simulink model "imu_pitch_cal_sim"  (Simulink 9.0)
settings: Solver=FixedStepDiscrete  StartTime=start_time  StopTime=stop_time  FixedStep=0.020  RelTol=1e-3  EnableMultiTasking=on
InitFcn:
  | imu_pitch_cal_sim_init
values from neighbouring files (symbols this model uses):
  imuX = WeighDebug_TOAeef_imu_accelX_t27    [extra_tip_sim_init.m]    (also in imu_pitch_cal_sim_init.m = WeighDebug_TOAeef_imu_accelX_t194)
  imuY = WeighDebug_TOAeef_imu_accelY_t27    [extra_tip_sim_init.m]    (also in imu_pitch_cal_sim_init.m = WeighDebug_TOAeef_imu_accelY_t194)
  imuZ = WeighDebug_TOAeef_imu_accelZ_t27    [extra_tip_sim_init.m]    (also in imu_pitch_cal_sim_init.m = WeighDebug_TOAeef_imu_accelZ_t194)
  liftAngle = WeighDebug_TOAlift_angle_t27    [extra_tip_sim_init.m]    (also in imu_pitch_cal_sim_init.m = WeighDebug_TOAlift_angle_t194)
  liftCylLength = WeighDebug_LiftCylNormLen_t27    [extra_tip_sim_init.m]    (also in imu_pitch_cal_sim_init.m = WeighDebug_LiftCylLenghtNorm_Val_t194)
  liftCylPress = WeighDebug_LiftCylPres_t27    [extra_tip_sim_init.m]    (also in imu_pitch_cal_sim_init.m = WeighDebug_LiftCylPres_t194)
  s1c1 = 515    [imu_pitch_cal_sim_init.m]
  s1c2 = 548    [imu_pitch_cal_sim_init.m]
  s1c3 = 579    [imu_pitch_cal_sim_init.m]
  s2c1 = s1c3 + 1    (= 580)    [imu_pitch_cal_sim_init.m]
  s2c2 = 616    [imu_pitch_cal_sim_init.m]
  s2c3 = 646    [imu_pitch_cal_sim_init.m]
  steerAng = WeighDebug_TOAsteering_angle_t27    [extra_tip_sim_init.m]    (also in imu_pitch_cal_sim_init.m = WeighDebug_TOAsteering_angle_t194)
  tiltExt = WeighDebug_TOAtilt_extension_t27    [extra_tip_sim_init.m]    (also in imu_pitch_cal_sim_init.m = WeighDebug_TOAtilt_extension_t194)
  tiltHePress = WeighDebug_TOAtilt_he_pressure_t27    [extra_tip_sim_init.m]    (also in imu_pitch_cal_sim_init.m = WeighDebug_TOAtilt_he_pressure_t194)
  tiltRePress = WeighDebug_TOAtilt_re_pressure_t27    [extra_tip_sim_init.m]    (also in imu_pitch_cal_sim_init.m = WeighDebug_TOAtilt_re_pressure_t194)
  time = t27    [extra_tip_sim_init.m]    (also in imu_pitch_cal_sim_init.m = t194)
  time2 = t27    [extra_tip_sim_init.m]    (also in imu_pitch_cal_sim_init.m = t194)
undefined symbols (not defined in the file or in its folder): g, timestep, toa_appNumber, toa_imu_lpf_cutoff_hz, toa_imuBasicOrient, toa_liftBoreDia, toa_tiltBoreDia, toa_tiltNumCyl, toa_tiltRodDia, toa_toolBcLength
libraries: simulink x10, simulink_extras x2, lib_CATutils_Filters_1Pole_LowPass x2, lib_CATutils_Override x1, lib_imuCal x1
settings Model: LogicAnalyzerSignalOrdering=5dd0029d-0573-49e1-b82a-316668c0f863,9c1653df-ca6c-4435-bc59-59c042f1a04b,b085631a-3729-4051-976c-78eb5fade8d3,7d46beec-13ab-48f4-a3cd-fd0effd7abe8,b6a03e28-23cb-43f9-a248-fda54d9653ab,a37efb6f-6706-4435-ba35-0122ce8219fd,a8a2ce2a-5a46-45c1-9d46-6a4d6193dbf9,5d366e23-9e16-40ab-92ec-e6241a047015,b6cb7851-fc42-42d8-ba93-f76abef1ebeb,7eca61fc-1cd1-4022-a45b-67ff63c6626d,6142d480-2c12-41e6-bc69-adb81a4771c4,b3c5c01d-7cb6-4bb7-bbe8-a848e78f78ed,24d79649-15d2-4718-8ed2-926b01c05a24,d8f024a4-d935-44db-a83c-243ca19a82d6,456d51b4-31c5-4d8b-9e4a-36f8ba5986a5,e5bf8900-4f4f-4702-ba55-200edadc7652,670c9483-bb58-4bfd-81ee-4bca25119f9a,78d642a3-b1b9-4e6b-84df-a8ec2d1c8fc5,fb89492d-1250-4bf5-972c-88d3c591c784,e773cc5f-bf5a-4589-b78e-aa1b72e66aaf,7a194ec3-8c67-49e0-a814-e64707b03eab,5e584c15-33ad-4c90-aebe-4c0d8ccecd57,a748872e-ecb8-4d69-a457-438b54df085b,bf746cf6-b149-4b19-87a9-88a499d409ce,04501ed4-9feb-42f8-8fc5-352602800299,46692b40-c2fd-4c0a-8a50-25bd1b341a8a,945a29ba-1fc8-4fc9-9c14-24f1e94ed818  MinMaxOverflowLogging=MinMaxAndOverflow  Creator=gulamhs  LastModifiedBy=CurriSD
settings DataIOCC: ExternalInput=[t,u]  SaveCompleteFinalSimState=on  SaveFormat=StructureWithTime  SaveOutput=off  SignalLogging=off  DSMLogging=off  SaveTime=off
settings OptimizationCC: DefaultParameterBehavior=Inlined  InlineInvariantSignals=on  EnhancedBackFolding=on  StrengthReduction=on  BitfieldContainerType=uchar_T  PassReuseOutputArgsAs=Individual arguments  ExpressionDepthLimit=2147483647  EfficientFloat2IntCast=on
settings DebuggingCC: SignalInfNanChecking=warning  SignalRangeChecking=error  ReadBeforeWriteMsg=EnableAllAsError  WriteAfterWriteMsg=EnableAllAsError  WriteAfterReadMsg=EnableAllAsError  AlgebraicLoopMsg=error  ArtificialAlgebraicLoopMsg=error  SaveWithDisabledLinksMsg=error  SaveWithParameterizedLinksMsg=error  UnderspecifiedInitializationDetection=Simplified  MergeDetectMultiDrivingBlocksExec=error  BlockPriorityViolationMsg=error  SolverPrmCheckMsg=error  InheritedTsInSrcMsg=none  TasksWithSamePriorityMsg=error  SigSpecEnsureSampleTimeMsg=error  CheckMatrixSingularityMsg=error  IntegerOverflowMsg=error  ParameterUnderflowMsg=error  ParameterPrecisionLossMsg=none  FixptConstUnderflowMsg=error  FixptConstOverflowMsg=error  UnderSpecifiedDataTypeMsg=error  FcnCallInpInsideContextMsg=warning  UnconnectedInputMsg=error  UnconnectedOutputMsg=error  UnconnectedLineMsg=error  SFcnCompatibilityMsg=error  FrameProcessingCompatibilityMsg=warning  UniqueDataStoreMsg=error  BusObjectLabelMismatch=error  RootOutportRequireBusObject=error  AssertControl=DisableAll  ModelReferenceIOMsg=error  ModelReferenceVersionMismatchMessage=warning  ModelReferenceIOMismatchMessage=error  UnknownTsInhSupMsg=error  ModelReferenceDataLoggingMessage=error  StateNameClashWarn=warning  SimStateInterfaceChecksumMismatchMsg=error  StrictBusMsg=ErrorOnBusTreatedAsVector  BusNameAdapt=ErrorWithoutRepair  NonBusSignalsTreatedAsBus=error  SFInvalidInputDataAccessInChartInitDiag=error  SFNoUnconditionalDefaultTransitionDiag=error  SFTransitionOutsideNaturalParentDiag=error  SFUnreachableExecutionPathDiag=error  SFUndirectedBroadcastEventsDiag=error  SFExecutionAtInitializationDiag=warning  IntegerSaturationMsg=error
settings HardwareCC: ProdBitPerLong=64  ProdBitPerPointer=64  ProdBitPerSizeT=64  ProdBitPerPtrDiffT=64  ProdLargestAtomicInteger=Integer  ProdLargestAtomicFloat=Float  ProdIntDivRoundTo=Zero  ProdEndianess=LittleEndian  ProdWordSize=64  ProdHWDeviceType=Intel->x86-64 (Linux 64)
settings ModelReferenceCC: ParallelModelReferenceMATLABWorkerInit=Load Top Model  PropagateSignalLabelsOutOfModel=on
settings SFSimCC: SimUserIncludeDirs=..\c_src  SFSimEcho=off  SimGenImportedTypeDefs=on  MATLABDynamicMemAlloc=off
settings SFSimCC: SimUserSources=|
  | ../c_src/tipoff_assist.c
  | ../c_src/tipoff_assist_950_14A_HL.c
  | ../c_src/tipoff_assist_950_14A_LOG.c
  | ../c_src/tipoff_assist_950_14A_STD.c
  | ../c_src/tipoff_assist_950_14A_Z_HL.c
  | ../c_src/tipoff_assist_950_14A_Z_LOG.c
  | ../c_src/tipoff_assist_950_14A_Z_STD.c
  | ../c_src/tipoff_assist_962_14A_HL.c
  | ../c_src/tipoff_assist_962_14A_LOG.c
  | ../c_src/tipoff_assist_962_14A_STD.c
  | ../c_src/tipoff_assist_962_14A_Z_HL.c
  | ../c_src/tipoff_assist_962_14A_Z_STD.c
  | ../c_src/tipoff_assist_966_14A_HL.c
  | ../c_src/tipoff_assist_966_14A_LOG.c
  | ../c_src/tipoff_assist_966_14A_STD.c
  | ../c_src/tipoff_assist_972_14A_HL.c
  | ../c_src/tipoff_assist_972_14A_STD.c
  | ../c_src/tipoff_assist_972_14A_SL.c
  | ../c_src/tipoff_assist_980_14A_BLK.c
  | ../c_src/tipoff_assist_980_14A_HL.c
  | ../c_src/tipoff_assist_980_14A_HVY.c
  | ../c_src/tipoff_assist_980_14A_LOG.c
  | ../c_src/tipoff_assist_980_14A_STD.c
  | ../c_src/tipoff_assist_982_14A_HL.c
  | ../c_src/tipoff_assist_982_14A_LOG.c
  | ../c_src/tipoff_assist_982_14A_STD.c
settings RTWCC: SystemTargetFile=cat_PkgArch.tlc  GenCodeOnly=on  GenerateMakefile=off  TemplateMakefile=cat_PkgArch_default_tmf  Description=R7a CAT Package Architecture Code Generation.  GenerateReport=on  RTWUseSimCustomCode=on  CustomInclude=..\c_src  CodeProfilingSaveOptions=AllData  GenerateTraceReport=on  GenerateTraceReportSl=on  GenerateTraceReportSf=on  GenerateTraceReportEml=on  GenerateWebview=on  GenerateCodeMetricsReport=on  GenerateCodeReplacementReport=on
settings RTWCC: CustomSource=|
  | ../c_src/tipoff_assist.c
  | ../c_src/tipoff_assist_950_14A_HL.c
  | ../c_src/tipoff_assist_950_14A_LOG.c
  | ../c_src/tipoff_assist_950_14A_STD.c
  | ../c_src/tipoff_assist_950_14A_Z_HL.c
  | ../c_src/tipoff_assist_950_14A_Z_LOG.c
  | ../c_src/tipoff_assist_950_14A_Z_STD.c
  | ../c_src/tipoff_assist_962_14A_HL.c
  | ../c_src/tipoff_assist_962_14A_LOG.c
  | ../c_src/tipoff_assist_962_14A_STD.c
  | ../c_src/tipoff_assist_962_14A_Z_HL.c
  | ../c_src/tipoff_assist_962_14A_Z_STD.c
  | ../c_src/tipoff_assist_966_14A_HL.c
  | ../c_src/tipoff_assist_966_14A_LOG.c
  | ../c_src/tipoff_assist_966_14A_STD.c
  | ../c_src/tipoff_assist_972_14A_HL.c
  | ../c_src/tipoff_assist_972_14A_STD.c
  | ../c_src/tipoff_assist_972_14A_SL.c
  | ../c_src/tipoff_assist_980_14A_BLK.c
  | ../c_src/tipoff_assist_980_14A_HL.c
  | ../c_src/tipoff_assist_980_14A_HVY.c
  | ../c_src/tipoff_assist_980_14A_LOG.c
  | ../c_src/tipoff_assist_980_14A_STD.c
  | ../c_src/tipoff_assist_982_14A_HL.c
  | ../c_src/tipoff_assist_982_14A_LOG.c
  | ../c_src/tipoff_assist_982_14A_STD.c
settings CodeAppCC: ForceParamTrailComments=on  IgnoreCustomStorageClasses=off  MaxIdLength=63  OperatorAnnotations=on  SimulinkDataObjDesc=on  SFDataObjDesc=on  MATLABFcnDesc=on  MangleLength=4  CustomSymbolStrType=$N$R$M  InsertBlockDesc=on  MATLABSourceComments=on  InternalIdentifier=Classic  ReqsInCode=on  UseSimReservedNames=on
settings STFCustomTargetCC: UtilityFuncGeneration=Shared location  MultiwordTypeDef=User defined  IncludeMdlTerminateFcn=off  CombineOutputUpdateFcns=on  SuppressErrorStatus=on  ERTCustomFileBanners=on  SupportAbsoluteTime=off  MultiInstanceERTCode=on  CodeInterfacePackaging=Reusable function  SupportComplex=off  SupportContinuousTime=off  SupportNonInlinedSFcns=off  RemoveResetFunc=on  SupportVariableSizeSignals=on  ParenthesesLevel=Maximum  MATLABClassNameForMDSCustomization=Simulink.SoftwareTarget.ERTCustomization  GRTInterface=off  GenerateSharedConstants=off  SystemTargetFile=cat_PkgArch.tlc
settings ERTTargetCC: UtilityFuncGeneration=Shared location  MultiwordTypeDef=User defined  MultiwordLength=2048  ParMdlRefBuildCompliant=off  CompOptLevelCompliant=off  ConcurrentExecutionCompliant=off  IncludeMdlTerminateFcn=off  SuppressErrorStatus=on  SupportAbsoluteTime=off  MultiInstanceERTCode=on  CodeInterfacePackaging=Reusable function  SupportComplex=off  SupportVariableSizeSignals=on  ParenthesesLevel=Maximum  ModelStepFunctionPrototypeControlCompliant=off  CPPClassGenCompliant=off  UseToolchainInfoCompliant=off  GenerateSharedConstants=off  MultiInstanceErrorCode=None  ERTSrcFileBannerTemplate=cat_code_template.cgt  ERTHdrFileBannerTemplate=cat_code_template.cgt  ERTDataSrcFileTemplate=cat_code_template.cgt  ERTDataHdrFileTemplate=cat_code_template.cgt  ERTCustomFileTemplate=cat_PkgArch_CFP.tlc  SuppressUnreachableDefaultCases=off  EnableUserReplacementTypes=on
settings MATStruct: int32=int32_t  int16=int16_t  int8=int8_t  uint32=uint32_t  uint16=uint16_t  uint8=uint8_t
settings CustomProperty: Value=Development
settings EnumStrPairs: String=Development
settings ConfigComp: CovScope=Subsystem  CovPath=/Chart1  CovMetricSettings=r  CovHtmlReporting=off  CovSaveCumulativeToWorkspaceVar=off  CovSaveSingleToWorkspaceVar=off  CovExternalEMLEnable=on

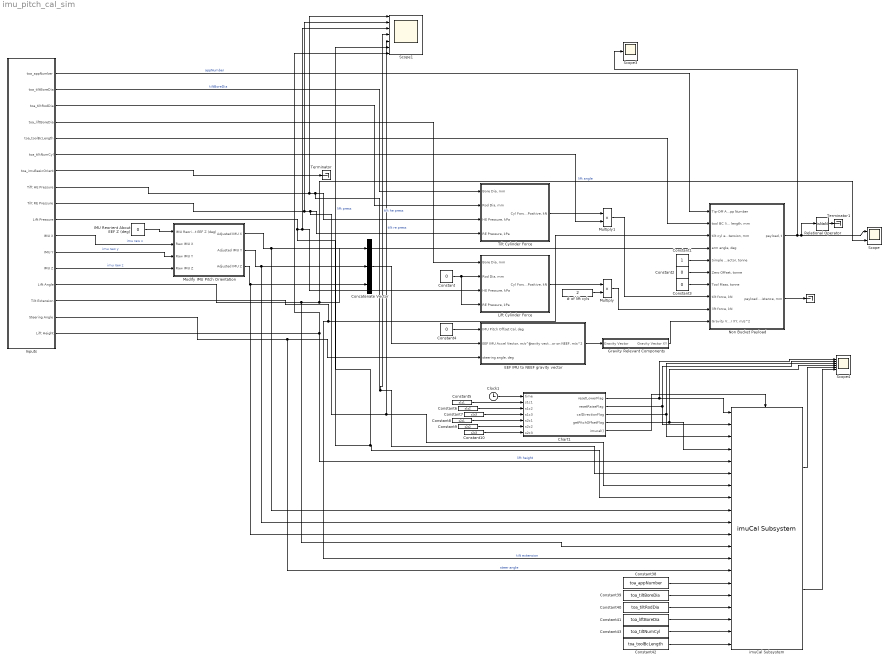
== system imu_pitch_cal_sim ==
  " " : Terminator
  # of lift cyls : Constant  Value=2  OutDataTypeStr=single
  Chart1 : Stateflow chart  TreatAsAtomicUnit=on
  Clock1 : Clock
      settings: Decimation=1000
  Concatenate Vector : Concatenate  NumInputs=3  Mode=Multidimensional array
  Constant : Constant  Value=0  OutDataTypeStr=Inherit: Inherit via back propagation
  Constant1 : Constant  OutDataTypeStr=single
  Constant10 : Constant  Value=s2c3
  Constant2 : Constant  Value=0  OutDataTypeStr=Inherit: Inherit via back propagation
  Constant3 : Constant  Value=0  OutDataTypeStr=Inherit: Inherit via back propagation
  Constant38 : Constant  Value=toa_appNumber  OutDataTypeStr=uint32
  Constant39 : Constant  Value=toa_tiltBoreDia  OutDataTypeStr=single
  Constant4 : Constant  Value=0  OutDataTypeStr=single
  Constant40 : Constant  Value=toa_tiltRodDia  OutDataTypeStr=single
  Constant41 : Constant  Value=toa_liftBoreDia  OutDataTypeStr=single
  Constant42 : Constant  Value=toa_toolBcLength  OutDataTypeStr=single
  Constant43 : Constant  Value=toa_tiltNumCyl  OutDataTypeStr=uint8
  Constant5 : Constant  Value=s1c1
  Constant6 : Constant  Value=s1c2
  Constant7 : Constant  Value=s1c3
  Constant8 : Constant  Value=s2c1
  Constant9 : Constant  Value=s2c2
  EEF IMU to NEEF gravity vector : Subsystem
  Gravity Relevant Components : Subsystem
  IMU Reorient About EEF Z (deg) : Constant  Value=0  OutDataTypeStr=single
  "Inputs " : Subsystem
  Lift Cylinder Force : Subsystem
  Modify IMU Pitch Orientation : Subsystem
  Multiply : Product  SaturateOnIntegerOverflow=on  RndMeth=Zero  InputSameDT=on  OutDataTypeStr=Inherit: Same as first input
  Multiply1 : Product  SaturateOnIntegerOverflow=on  RndMeth=Zero  InputSameDT=on  OutDataTypeStr=Inherit: Same as first input
  Non Bucket Payload : Subsystem
  Relational Operator : RelationalOperator  Operator=isNaN  OutDataTypeStr=boolean  RndMeth=Simplest
  Scope : Scope  NumInputPorts=2
  Scope1 : Scope  NumInputPorts=7
  Scope3 : Scope
  Scope4 : Scope  NumInputPorts=6
  Terminator : Terminator
  Terminator1 : Terminator
  Tilt Cylinder Force : Subsystem
  imuCal Subsystem : lib_imuCal/imuCal Subsystem
  wires:
  Multiply/1 -> Non Bucket Payload/9("lift force, kN")
  Non Bucket Payload/1("payload, t") -> Scope3/1, Scope/1, Relational Operator/1
  Multiply1/1 -> Non Bucket Payload/8("tilt force, kN")
  "Inputs "/6(toa_tiltNumCyl) -> Multiply1/2
  EEF IMU to NEEF gravity vector/1("gravity vector on NEEF, m/s^2") -> Gravity Relevant Components/1(Gravity Vector)
  Lift Cylinder Force/1("Cyl Force, Compression Positive, kN") -> Multiply/1
  Non Bucket Payload/2("payload distance, mm") -> " "/1
  # of lift cyls/1 -> Multiply/2
  Tilt Cylinder Force/1("Cyl Force, Compression Positive, kN") -> Multiply1/1
  Gravity Relevant Components/1(Gravity Vector XY) -> Non Bucket Payload/10("Gravity Vector XY, m/s^2")
  "Inputs "/1(toa_appNumber) -> Non Bucket Payload/1(Tip-Off Assist App Number)  "appNumber"
  "Inputs "/2(toa_tiltBoreDia) -> Tilt Cylinder Force/1("Bore Dia, mm")  "tiltBoreDia"
  "Inputs "/3(toa_tiltRodDia) -> Tilt Cylinder Force/2("Rod Dia, mm")
  "Inputs "/8(Tift HE Pressure) -> Scope1/1, Scope1/4, imuCal Subsystem/6, Tilt Cylinder Force/3("HE Pressure, kPa")  "tilt he press"
  "Inputs "/9(Tilt RE Pressure) -> Scope1/2, Scope1/5, imuCal Subsystem/7, Tilt Cylinder Force/4("RE Pressure, kPa")  "tilt re press"
  "Inputs "/4(toa_liftBoreDia) -> Lift Cylinder Force/1("Bore Dia, mm")
  "Inputs "/10(Lift Pressure) -> Scope1/6, imuCal Subsystem/8, Lift Cylinder Force/3("HE Pressure, kPa"), Scope1/3  "lift press"
  Constant/1 -> Lift Cylinder Force/4("RE Pressure, kPa"), Lift Cylinder Force/2("Rod Dia, mm")
  "Inputs "/11(IMU X) -> Modify IMU Pitch Orientation/2(Raw IMU X)  "imu raw x"
  Concatenate Vector/1 -> EEF IMU to NEEF gravity vector/2("EEF IMU Accel Vector, m/s^2")
  "Inputs "/16(Steering Angle) -> imuCal Subsystem/14, EEF IMU to NEEF gravity vector/3("steering angle, deg")  "steer angle"
  "Inputs "/15(Tilt Extension) -> imuCal Subsystem/13, Non Bucket Payload/3("tilt cyl extension, mm")  "tilt extension"
  "Inputs "/14(Lift Angle) -> imuCal Subsystem/12, Scope/2, Non Bucket Payload/4("arm angle, deg")  "lift angle"
  "Inputs "/7(toa_imuBasicOrient) -> Terminator/1
  "Inputs "/5(toa_toolBcLength) -> Non Bucket Payload/2("tool BC link length, mm")
  Constant1/1 -> Non Bucket Payload/5("Simple Cal Factor, tonne")
  Constant2/1 -> Non Bucket Payload/6("Zero Offset, tonne")
  Constant3/1 -> Non Bucket Payload/7("Tool Mass, tonne")
  Relational Operator/1 -> Terminator1/1
  Constant4/1 -> EEF IMU to NEEF gravity vector/1("IMU Pitch Offset Cal, deg")
  Chart1/1(resetLowerFlag) -> Scope4/1, imuCal Subsystem/1
  Chart1/3(calDirectionFlag) -> Scope4/3, imuCal Subsystem/3
  Chart1/4(getPitchOffsetFlag) -> Scope4/4, imuCal Subsystem/4
  Clock1/1 -> Chart1/1(time)
  "Inputs "/17(Lift Height) -> Scope1/7, imuCal Subsystem/5  "lift height"
  Chart1/2(resetRaiseFlag) -> Scope4/2, imuCal Subsystem/2
  Chart1/5(imucal()) -> imuCal Subsystem/Trigger
  imuCal Subsystem/1 -> Scope4/5
  Constant5/1 -> Chart1/2(s1c1)
  Constant6/1 -> Chart1/3(s1c2)
  Constant7/1 -> Chart1/4(s1c3)
  Constant8/1 -> Chart1/5(s2c1)
  Constant9/1 -> Chart1/6(s2c2)
  Constant10/1 -> Chart1/7(s2c3)
  Constant38/1 -> imuCal Subsystem/15
  Constant39/1 -> imuCal Subsystem/16
  Constant40/1 -> imuCal Subsystem/17
  Constant41/1 -> imuCal Subsystem/18
  Constant43/1 -> imuCal Subsystem/19
  Constant42/1 -> imuCal Subsystem/20
  IMU Reorient About EEF Z (deg)/1 -> Modify IMU Pitch Orientation/1(IMU Reorient EEF Z (deg))
  "Inputs "/12(IMU Y) -> Modify IMU Pitch Orientation/3(Raw IMU Y)  "imu raw y"
  "Inputs "/13(IMU Z) -> Modify IMU Pitch Orientation/4(Raw IMU Z)  "imu raw z"
  Modify IMU Pitch Orientation/1(Adjusted IMU X) -> imuCal Subsystem/9, Concatenate Vector/1
  Modify IMU Pitch Orientation/2(Adjusted IMU Y) -> imuCal Subsystem/10, Concatenate Vector/2
  Modify IMU Pitch Orientation/3(Adjusted IMU Z) -> imuCal Subsystem/11, Concatenate Vector/3
  imuCal Subsystem/2 -> Scope4/6

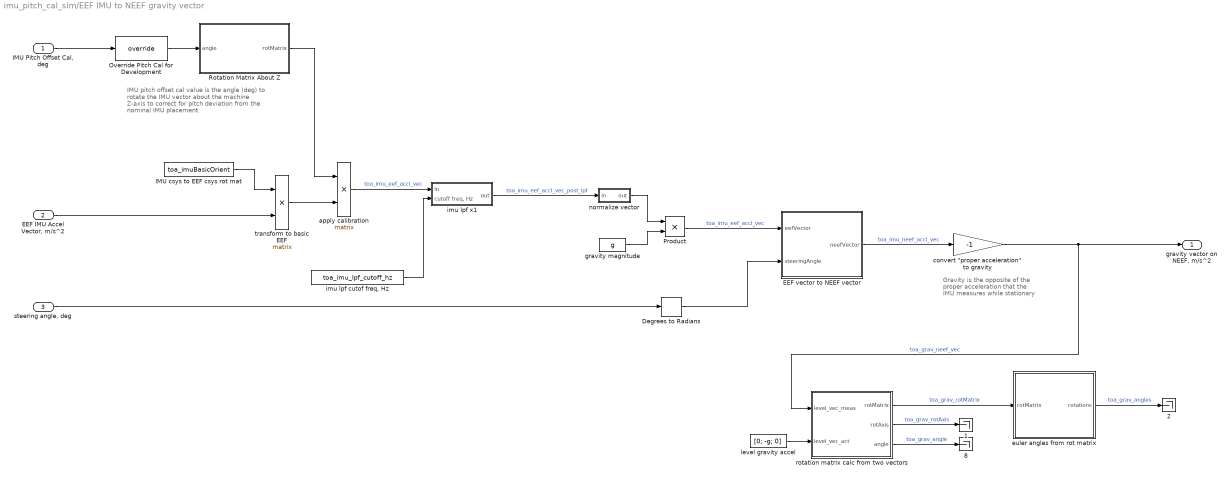
== system imu_pitch_cal_sim/EEF IMU to NEEF gravity vector ==
  note: Gravity is the opposite of the proper acceleration that the IMU measures while stationary
  note: IMU pitch offset cal value is the angle (deg) to rotate the IMU vector about the machine Z-axis to correct for pitch deviation from the nominal IMU placement.
  "IMU Pitch Offset Cal, deg" : Inport
  "EEF IMU Accel Vector, m/s^2" : Inport  Port=2
  "steering angle, deg" : Inport  Port=3
  " 1" : Terminator
  " 2" : Terminator
  " 8" : Terminator
  Degrees to Radians : simulink_extras/Transformations/Degrees to Radians
  EEF vector to NEEF vector : MATLAB Function  TreatAsAtomicUnit=on
  IMU csys to EEF csys rot mat : Constant  Value=toa_imuBasicOrient  VectorParams1D=off  OutDataTypeStr=single  SampleTime=-1
  Override Pitch Cal for Development : lib_CATutils_Override/override  ovType=OV if OV ~= Pass  extOV=off  ov_value=toa_imuCalPitchAngOv  extPass=off  pass_value=360  extRange=off  ov_max=100  ov_min=1  extCond=off  ov_cond=toa_imuCalPitchAngOv  extTF=off  ov_TrueComp=1  ov_FalseComp=2
  Product : Product  Inputs=**  OutDataTypeStr=Inherit: Same as first input
  Rotation Matrix About Z : MATLAB Function  TreatAsAtomicUnit=on
  apply calibration : Product  Multiplication=Matrix(*)  SaturateOnIntegerOverflow=on  RndMeth=Zero  OutDataTypeStr=Inherit: Same as first input
  "convert \"proper acceleration\" to gravity" : Gain  Gain=-1  SaturateOnIntegerOverflow=on  OutDataTypeStr=Inherit: Same as input  ParamDataTypeStr=Inherit: Same as input
  euler angles from rot matrix : MATLAB Function  TreatAsAtomicUnit=on
  gravity magnitude : Constant  Value=g  OutDataTypeStr=single  SampleTime=timestep
  "imu lpf cutof freq, Hz" : Constant  Value=toa_imu_lpf_cutoff_hz  OutDataTypeStr=single  SampleTime=timestep
  imu lpf x1 : Subsystem
  level gravity accel : Constant  Value=[0; -g; 0]  OutDataTypeStr=single  SampleTime=-1
  normalize vector : Subsystem
  rotation matrix calc from two vectors : MATLAB Function  TreatAsAtomicUnit=on
  transform to basic EEF : Product  Multiplication=Matrix(*)  SaturateOnIntegerOverflow=on  RndMeth=Zero  OutDataTypeStr=Inherit: Same as first input
  "gravity vector on NEEF, m/s^2" : Outport
  wires:
  "IMU Pitch Offset Cal, deg"/1 -> Override Pitch Cal for Development/1
  euler angles from rot matrix/1(rotations) -> " 2"/1  "toa_grav_angles"
  "imu lpf cutof freq, Hz"/1 -> imu lpf x1/2("cutoff freq, Hz")
  Degrees to Radians/1 -> EEF vector to NEEF vector/2(steeringAngle)
  Product/1 -> EEF vector to NEEF vector/1(eefVector)  "toa_imu_eef_accl_vec"
  "steering angle, deg"/1 -> Degrees to Radians/1
  EEF vector to NEEF vector/1(neefVector) -> "convert \"proper acceleration\" to gravity"/1  "toa_imu_neef_accl_vec"
  normalize vector/1(out) -> Product/1
  imu lpf x1/1(out) -> normalize vector/1(in)  "toa_imu_eef_accl_vec_post_lpf"
  gravity magnitude/1 -> Product/2
  Override Pitch Cal for Development/1 -> Rotation Matrix About Z/1(angle)
  Rotation Matrix About Z/1(rotMatrix) -> apply calibration/1
  apply calibration/1 -> imu lpf x1/1(in)  "toa_imu_eef_accl_vec"
  transform to basic EEF/1 -> apply calibration/2
  IMU csys to EEF csys rot mat/1 -> transform to basic EEF/1
  "convert \"proper acceleration\" to gravity"/1 -> rotation matrix calc from two vectors/1(level_vec_meas), "gravity vector on NEEF, m/s^2"/1  "toa_grav_neef_vec"
  "EEF IMU Accel Vector, m/s^2"/1 -> transform to basic EEF/2
  rotation matrix calc from two vectors/1(rotMatrix) -> euler angles from rot matrix/1(rotMatrix)  "toa_grav_rotMatrix"
  rotation matrix calc from two vectors/2(rotAxis) -> " 1"/1  "toa_grav_rotAxis"
  rotation matrix calc from two vectors/3(angle) -> " 8"/1  "toa_grav_angle"
  level gravity accel/1 -> rotation matrix calc from two vectors/2(level_vec_act)

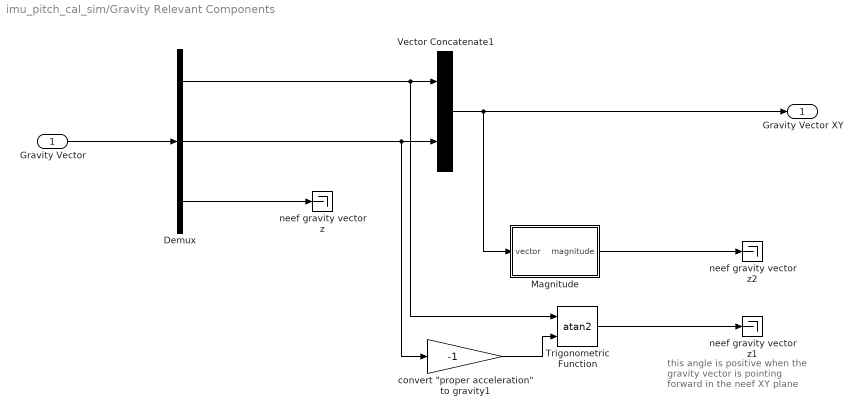
== system imu_pitch_cal_sim/Gravity Relevant Components ==
  note: this angle is positive when the gravity vector is pointing forward in the neef XY plane
  Gravity Vector : Inport
  " neef gravity vector z" : Terminator
  " neef gravity vector z1" : Terminator
  " neef gravity vector z2" : Terminator
  Demux : Demux  Outputs=3
  Magnitude : Subsystem
  Trigonometric Function : Trigonometry  Operator=atan2  OutputSignalType=real
  Vector Concatenate1 : Concatenate  Mode=Multidimensional array
  "convert \"proper acceleration\" to gravity1" : Gain  Gain=-1  SaturateOnIntegerOverflow=on  OutDataTypeStr=Inherit: Same as input  ParamDataTypeStr=Inherit: Same as input
  Gravity Vector XY : Outport
  wires:
  Gravity Vector/1 -> Demux/1
  Demux/2 -> "convert \"proper acceleration\" to gravity1"/1, Vector Concatenate1/2
  Demux/1 -> Trigonometric Function/1, Vector Concatenate1/1
  Magnitude/1(magnitude) -> " neef gravity vector z2"/1
  Trigonometric Function/1 -> " neef gravity vector z1"/1
  "convert \"proper acceleration\" to gravity1"/1 -> Trigonometric Function/2
  Demux/3 -> " neef gravity vector z"/1
  Vector Concatenate1/1 -> Magnitude/1(vector), Gravity Vector XY/1

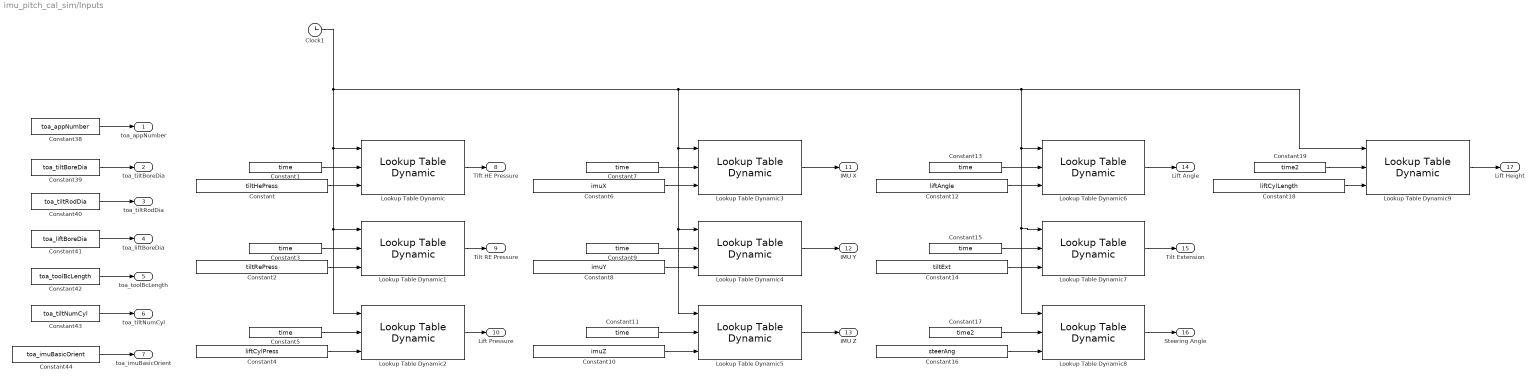
== system imu_pitch_cal_sim/Inputs  ==
  Clock1 : Clock
      settings: Decimation=1000
  Constant : Constant  Value=tiltHePress  SampleTime=timestep
  Constant{1,3,5,7,9,11,13,15} (8 alike) : Constant  Value=time  SampleTime=timestep
  Constant10 : Constant  Value=imuZ  SampleTime=timestep
  Constant12 : Constant  Value=liftAngle  SampleTime=timestep
  Constant14 : Constant  Value=tiltExt  SampleTime=timestep
  Constant16 : Constant  Value=steerAng  SampleTime=timestep
  Constant17 : Constant  Value=time2  SampleTime=timestep
  Constant18 : Constant  Value=liftCylLength  SampleTime=timestep
  Constant19 : Constant  Value=time2  SampleTime=timestep
  Constant2 : Constant  Value=tiltRePress  SampleTime=timestep
  Constant38 : Constant  Value=toa_appNumber  OutDataTypeStr=uint32
  Constant39 : Constant  Value=toa_tiltBoreDia  OutDataTypeStr=single
  Constant4 : Constant  Value=liftCylPress  SampleTime=timestep
  Constant40 : Constant  Value=toa_tiltRodDia  OutDataTypeStr=single
  Constant41 : Constant  Value=toa_liftBoreDia  OutDataTypeStr=single
  Constant42 : Constant  Value=toa_toolBcLength  OutDataTypeStr=single
  Constant43 : Constant  Value=toa_tiltNumCyl  OutDataTypeStr=single
  Constant44 : Constant  Value=toa_imuBasicOrient
  Constant6 : Constant  Value=imuX  SampleTime=timestep
  Constant8 : Constant  Value=imuY  SampleTime=timestep
  Lookup Table Dynamic{,1..9} (10 alike) : simulink/Lookup Tables/Lookup Table Dynamic  LookUpMeth=Interpolation-Use End Values  OutDataType=fixdt('single')  OutScaling=[]  OutputDataTypeScalingMode=Specify via dialog  OutDataTypeStr=single  DoSatur=off
      settings: SourceProductName=Simulink
  toa_appNumber : Outport  SampleTime=timestep
  toa_tiltBoreDia : Outport  Port=2  SampleTime=timestep
  toa_tiltRodDia : Outport  Port=3  SampleTime=timestep
  toa_liftBoreDia : Outport  Port=4  SampleTime=timestep
  toa_toolBcLength : Outport  Port=5  SampleTime=timestep
  toa_tiltNumCyl : Outport  Port=6  SampleTime=timestep
  toa_imuBasicOrient : Outport  Port=7  SampleTime=timestep
  Tift HE Pressure : Outport  Port=8  SampleTime=timestep
  Tilt RE Pressure : Outport  Port=9  SampleTime=timestep
  Lift Pressure : Outport  Port=10  SampleTime=timestep
  IMU X : Outport  Port=11  SampleTime=timestep
  IMU Y : Outport  Port=12  SampleTime=timestep
  IMU Z : Outport  Port=13  SampleTime=timestep
  Lift Angle : Outport  Port=14  SampleTime=timestep
  Tilt Extension : Outport  Port=15  SampleTime=timestep
  Steering Angle : Outport  Port=16  SampleTime=timestep
  Lift Height : Outport  Port=17  SampleTime=timestep
  wires:
  Constant17/1 -> Lookup Table Dynamic8/2
  Constant13/1 -> Lookup Table Dynamic6/2
  Lookup Table Dynamic6/1 -> Lift Angle/1
  Lookup Table Dynamic5/1 -> IMU Z/1
  Constant/1 -> Lookup Table Dynamic/3
  Lookup Table Dynamic2/1 -> Lift Pressure/1
  Constant3/1 -> Lookup Table Dynamic1/2
  Constant2/1 -> Lookup Table Dynamic1/3
  Constant8/1 -> Lookup Table Dynamic4/3
  Constant9/1 -> Lookup Table Dynamic4/2
  Constant12/1 -> Lookup Table Dynamic6/3
  Constant15/1 -> Lookup Table Dynamic7/2
  Lookup Table Dynamic7/1 -> Tilt Extension/1
  Lookup Table Dynamic8/1 -> Steering Angle/1
  Constant16/1 -> Lookup Table Dynamic8/3
  Constant11/1 -> Lookup Table Dynamic5/2
  Constant14/1 -> Lookup Table Dynamic7/3
  Constant6/1 -> Lookup Table Dynamic3/3
  Lookup Table Dynamic/1 -> Tift HE Pressure/1
  Constant4/1 -> Lookup Table Dynamic2/3
  Lookup Table Dynamic3/1 -> IMU X/1
  Lookup Table Dynamic4/1 -> IMU Y/1
  Constant1/1 -> Lookup Table Dynamic/2
  Constant7/1 -> Lookup Table Dynamic3/2
  Constant5/1 -> Lookup Table Dynamic2/2
  Constant10/1 -> Lookup Table Dynamic5/3
  Lookup Table Dynamic1/1 -> Tilt RE Pressure/1
  Constant39/1 -> toa_tiltBoreDia/1
  Constant38/1 -> toa_appNumber/1
  Constant40/1 -> toa_tiltRodDia/1
  Constant41/1 -> toa_liftBoreDia/1
  Constant42/1 -> toa_toolBcLength/1
  Constant43/1 -> toa_tiltNumCyl/1
  Constant44/1 -> toa_imuBasicOrient/1
  Clock1/1 -> Lookup Table Dynamic/1, Lookup Table Dynamic1/1, Lookup Table Dynamic2/1, Lookup Table Dynamic6/1, Lookup Table Dynamic7/1, Lookup Table Dynamic8/1, Lookup Table Dynamic9/1, Lookup Table Dynamic3/1, Lookup Table Dynamic5/1, Lookup Table Dynamic4/1
  Lookup Table Dynamic9/1 -> Lift Height/1
  Constant19/1 -> Lookup Table Dynamic9/2
  Constant18/1 -> Lookup Table Dynamic9/3

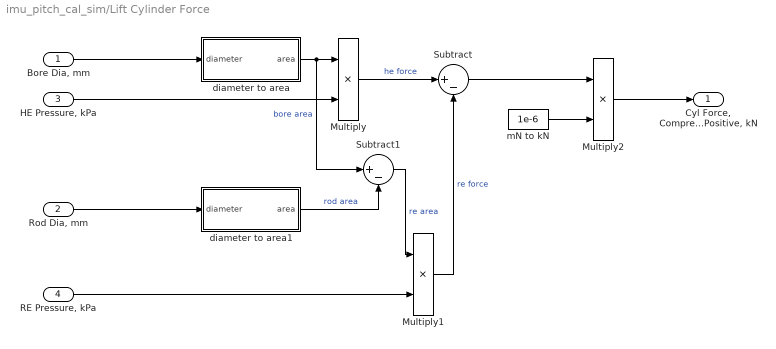
== system imu_pitch_cal_sim/Lift Cylinder Force ==
  "Bore Dia, mm" : Inport
  "Rod Dia, mm" : Inport  Port=2
  "HE Pressure, kPa" : Inport  Port=3
  "RE Pressure, kPa" : Inport  Port=4
  Multiply : Product  SaturateOnIntegerOverflow=on  RndMeth=Zero  InputSameDT=on  OutDataTypeStr=Inherit: Same as first input
  Multiply1 : Product  SaturateOnIntegerOverflow=on  RndMeth=Zero  InputSameDT=on  OutDataTypeStr=Inherit: Same as first input
  Multiply2 : Product  SaturateOnIntegerOverflow=on  RndMeth=Zero  InputSameDT=on  OutDataTypeStr=Inherit: Same as first input
  Subtract : Sum  Inputs=|+-  SaturateOnIntegerOverflow=on  InputSameDT=on  OutDataTypeStr=Inherit: Same as first input
  Subtract1 : Sum  Inputs=|+-  SaturateOnIntegerOverflow=on  InputSameDT=on  OutDataTypeStr=Inherit: Same as first input
  diameter to area : Subsystem
  diameter to area1 : Subsystem
  mN to kN : Constant  Value=1e-6  OutDataTypeStr=single
  "Cyl Force, Compression Positive, kN" : Outport
  wires:
  "HE Pressure, kPa"/1 -> Multiply/2
  Subtract/1 -> Multiply2/1
  "Bore Dia, mm"/1 -> diameter to area/1(diameter)
  Multiply1/1 -> Subtract/2  "re force"
  Multiply/1 -> Subtract/1  "he force"
  diameter to area/1(area) -> Subtract1/1, Multiply/1  "bore area"
  diameter to area1/1(area) -> Subtract1/2  "rod area"
  "RE Pressure, kPa"/1 -> Multiply1/2
  "Rod Dia, mm"/1 -> diameter to area1/1(diameter)
  Subtract1/1 -> Multiply1/1  "re area"
  mN to kN/1 -> Multiply2/2
  Multiply2/1 -> "Cyl Force, Compression Positive, kN"/1

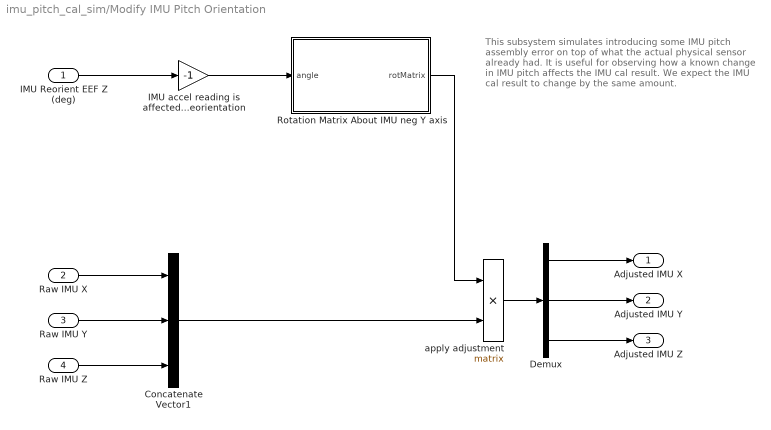
== system imu_pitch_cal_sim/Modify IMU Pitch Orientation ==
  note: This subsystem simulates introducing some IMU pitch assembly error on top of what the actual physical sensor already had. It is useful for observing how a known change in IMU pitch affects the IMU cal result. We expect the IMU cal result to change by the same amount.
  IMU Reorient EEF Z (deg) : Inport
  Raw IMU X : Inport  Port=2
  Raw IMU Y : Inport  Port=3
  Raw IMU Z : Inport  Port=4
  Concatenate Vector1 : Concatenate  NumInputs=3  Mode=Multidimensional array
  Demux : Demux  Outputs=3
  IMU accel reading is affected opposite of IMU body reorientation : Gain  Gain=-1
  Rotation Matrix About IMU neg Y axis : MATLAB Function  TreatAsAtomicUnit=on
  apply adjustment : Product  Multiplication=Matrix(*)  SaturateOnIntegerOverflow=on  RndMeth=Zero  OutDataTypeStr=Inherit: Same as first input
  Adjusted IMU X : Outport
  Adjusted IMU Y : Outport  Port=2
  Adjusted IMU Z : Outport  Port=3
  wires:
  Rotation Matrix About IMU neg Y axis/1(rotMatrix) -> apply adjustment/1
  apply adjustment/1 -> Demux/1
  Demux/1 -> Adjusted IMU X/1
  Demux/2 -> Adjusted IMU Y/1
  Demux/3 -> Adjusted IMU Z/1
  Raw IMU X/1 -> Concatenate Vector1/1
  Raw IMU Y/1 -> Concatenate Vector1/2
  IMU Reorient EEF Z (deg)/1 -> IMU accel reading is affected opposite of IMU body reorientation/1
  Raw IMU Z/1 -> Concatenate Vector1/3
  Concatenate Vector1/1 -> apply adjustment/2
  IMU accel reading is affected opposite of IMU body reorientation/1 -> Rotation Matrix About IMU neg Y axis/1(angle)

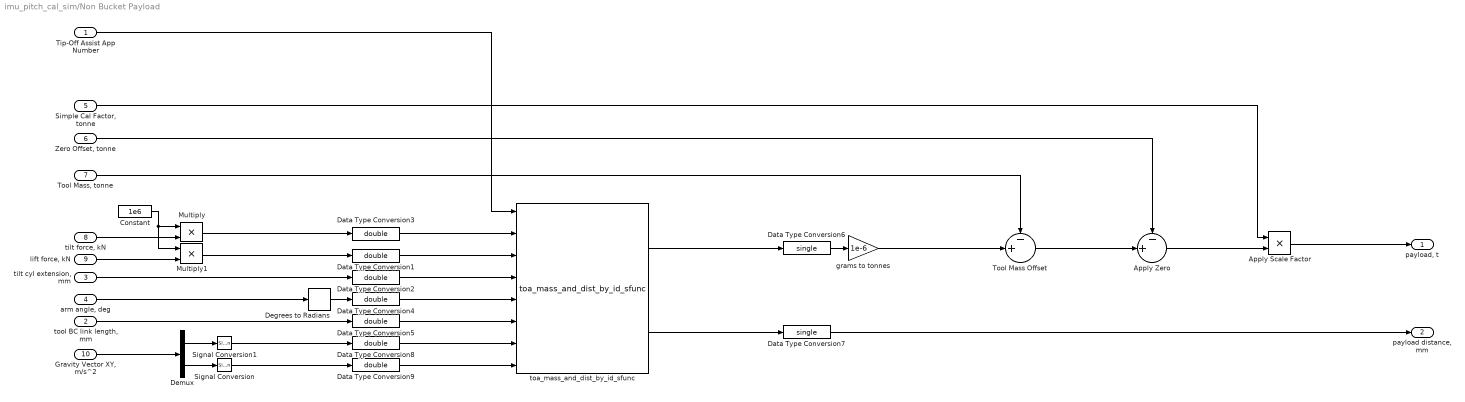
== system imu_pitch_cal_sim/Non Bucket Payload ==
  Tip-Off Assist App Number : Inport
  "tool BC link length, mm" : Inport  Port=2
  "tilt cyl extension, mm" : Inport  Port=3
  "arm angle, deg" : Inport  Port=4
  "Simple Cal Factor, tonne" : Inport  Port=5
  "Zero Offset, tonne" : Inport  Port=6
  "Tool Mass, tonne" : Inport  Port=7
  "tilt force, kN" : Inport  Port=8
  "lift force, kN" : Inport  Port=9
  "Gravity Vector XY, m/s^2" : Inport  Port=10
  Apply Scale Factor : Product
  Apply Zero : Sum  Inputs=-+|  SaturateOnIntegerOverflow=on  InputSameDT=on  OutDataTypeStr=Inherit: Same as first input
  Constant : Constant  Value=1e6  OutDataTypeStr=single
  Data Type Conversion{1..5,8..9} (7 alike) : DataTypeConversion  OutDataTypeStr=double  SaturateOnIntegerOverflow=on  RndMeth=Zero
      settings: AttributesFormatString=Output Data Type: %<OutDataTypeStr>\n
  Data Type Conversion6 : DataTypeConversion  OutDataTypeStr=single  SaturateOnIntegerOverflow=on  RndMeth=Zero
      settings: AttributesFormatString=Output Data Type: %<OutDataTypeStr>\n
  Data Type Conversion7 : DataTypeConversion  OutDataTypeStr=single  SaturateOnIntegerOverflow=on  RndMeth=Zero
      settings: AttributesFormatString=Output Data Type: %<OutDataTypeStr>\n
  Degrees to Radians : simulink_extras/Transformations/Degrees to Radians
  Demux : Demux  Outputs=2
  Multiply : Product  SaturateOnIntegerOverflow=on  RndMeth=Zero  InputSameDT=on  OutDataTypeStr=Inherit: Same as first input
  Multiply1 : Product  SaturateOnIntegerOverflow=on  RndMeth=Zero  InputSameDT=on  OutDataTypeStr=Inherit: Same as first input
  Signal Conversion : SignalConversion  OverrideOpt=on
  Signal Conversion1 : SignalConversion  OverrideOpt=on
  Tool Mass Offset : Sum  Inputs=-+|  SaturateOnIntegerOverflow=on  InputSameDT=on  OutDataTypeStr=Inherit: Same as first input
  grams to tonnes : Gain  Gain=1e-6  SaturateOnIntegerOverflow=on  OutDataTypeStr=Inherit: Same as input  ParamDataTypeStr=Inherit: Same as input
  toa_mass_and_dist_by_id_sfunc : S-Function  FunctionName=toa_mass_and_dist_by_id_sfunc  SFunctionDeploymentMode=off  EnableBusSupport=off  mask(Legacy Function){SFunctionSpec=void toa_mass_and_dist_by_id(uint32 u1, double u2, double u3, double u4, double u5, double u6, double u7, double u8, double y1[1], double y2[1]), ShowSpec=off}
      mask prompts: ShowSpec "Display function specification"
      mask help:
      | This block allows you to call the legacy functions specified by the following Legacy Code Tool definition:
      | def.SFunctionName = 'toa_mass_and_dist_by_id_sfunc';
      | def.OutputFcnSpec = 'void toa_mass_and_dist_by_id(uint32 u1, double u2, double u3, double u4, double u5, double u6, double u7, double u8, double y1[1], double y2[1])';
      | def.HeaderFiles = {'tipoff_assist.h'};
      | def.SourceFiles = {'tipoff_assist.c'};
      | def.IncPaths = {'./c_src'};
      mask Help: <p>This block was generated automatically by the Legacy Code Tool. For detailed help on this tool, call<a href="matlab:legacy_code('help')"> legacy_code('help')</a>.</p>
      mask Callback ShowSpec:
      | if strcmp(get_param(gcbh, 'ShowSpec'), 'on')
      |   set_param(gcbh, 'MaskDisplay', sprintf('fprintf(''%s'');', get_param(gcbh, 'SFunctionSpec')));
      | else
      |   set_param(gcbh, 'MaskDisplay', sprintf('fprintf(''%s'');', get_param(gcbh, 'FunctionName')));
      | end
      mask Display: fprintf('toa_mass_and_dist_by_id_sfunc');
  "payload, t" : Outport
  "payload distance, mm" : Outport  Port=2
  wires:
  Signal Conversion1/1 -> Data Type Conversion8/1
  Signal Conversion/1 -> Data Type Conversion9/1
  "tilt cyl extension, mm"/1 -> Data Type Conversion2/1
  Apply Scale Factor/1 -> "payload, t"/1
  Apply Zero/1 -> Apply Scale Factor/2
  "Simple Cal Factor, tonne"/1 -> Apply Scale Factor/1
  "Zero Offset, tonne"/1 -> Apply Zero/1
  Tool Mass Offset/1 -> Apply Zero/2
  Data Type Conversion3/1 -> toa_mass_and_dist_by_id_sfunc/2
  Data Type Conversion1/1 -> toa_mass_and_dist_by_id_sfunc/3
  Data Type Conversion2/1 -> toa_mass_and_dist_by_id_sfunc/4
  Data Type Conversion4/1 -> toa_mass_and_dist_by_id_sfunc/5
  Data Type Conversion5/1 -> toa_mass_and_dist_by_id_sfunc/6
  Data Type Conversion8/1 -> toa_mass_and_dist_by_id_sfunc/7
  Data Type Conversion9/1 -> toa_mass_and_dist_by_id_sfunc/8
  Tip-Off Assist App Number/1 -> toa_mass_and_dist_by_id_sfunc/1
  "tilt force, kN"/1 -> Multiply/2
  "lift force, kN"/1 -> Multiply1/2
  Constant/1 -> Multiply1/1, Multiply/1
  Data Type Conversion6/1 -> grams to tonnes/1
  Data Type Conversion7/1 -> "payload distance, mm"/1
  "Tool Mass, tonne"/1 -> Tool Mass Offset/1
  "Gravity Vector XY, m/s^2"/1 -> Demux/1
  grams to tonnes/1 -> Tool Mass Offset/2
  toa_mass_and_dist_by_id_sfunc/2 -> Data Type Conversion7/1
  toa_mass_and_dist_by_id_sfunc/1 -> Data Type Conversion6/1
  "tool BC link length, mm"/1 -> Data Type Conversion5/1
  Demux/2 -> Signal Conversion/1
  Demux/1 -> Signal Conversion1/1
  Multiply1/1 -> Data Type Conversion1/1
  Multiply/1 -> Data Type Conversion3/1
  "arm angle, deg"/1 -> Degrees to Radians/1
  Degrees to Radians/1 -> Data Type Conversion4/1

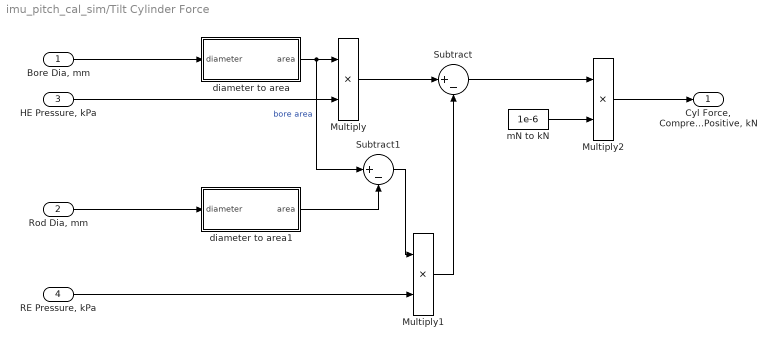
== system imu_pitch_cal_sim/Tilt Cylinder Force ==
  "Bore Dia, mm" : Inport
  "Rod Dia, mm" : Inport  Port=2
  "HE Pressure, kPa" : Inport  Port=3
  "RE Pressure, kPa" : Inport  Port=4
  Multiply : Product  SaturateOnIntegerOverflow=on  RndMeth=Zero  InputSameDT=on  OutDataTypeStr=Inherit: Same as first input
  Multiply1 : Product  SaturateOnIntegerOverflow=on  RndMeth=Zero  InputSameDT=on  OutDataTypeStr=Inherit: Same as first input
  Multiply2 : Product  SaturateOnIntegerOverflow=on  RndMeth=Zero  InputSameDT=on  OutDataTypeStr=Inherit: Same as first input
  Subtract : Sum  Inputs=|+-  SaturateOnIntegerOverflow=on  InputSameDT=on  OutDataTypeStr=Inherit: Same as first input
  Subtract1 : Sum  Inputs=|+-  SaturateOnIntegerOverflow=on  InputSameDT=on  OutDataTypeStr=Inherit: Same as first input
  diameter to area : Subsystem
  diameter to area1 : Subsystem
  mN to kN : Constant  Value=1e-6  OutDataTypeStr=single
  "Cyl Force, Compression Positive, kN" : Outport
  wires:
  "HE Pressure, kPa"/1 -> Multiply/2
  Subtract/1 -> Multiply2/1
  "Bore Dia, mm"/1 -> diameter to area/1(diameter)
  Multiply1/1 -> Subtract/2
  Multiply/1 -> Subtract/1
  diameter to area/1(area) -> Subtract1/1, Multiply/1  "bore area"
  diameter to area1/1(area) -> Subtract1/2
  "RE Pressure, kPa"/1 -> Multiply1/2
  "Rod Dia, mm"/1 -> diameter to area1/1(diameter)
  Subtract1/1 -> Multiply1/1
  mN to kN/1 -> Multiply2/2
  Multiply2/1 -> "Cyl Force, Compression Positive, kN"/1

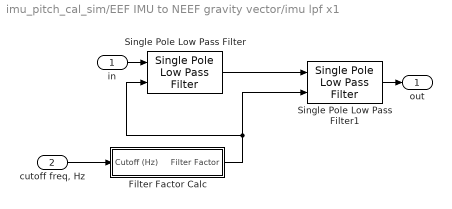
== system imu_pitch_cal_sim/EEF IMU to NEEF gravity vector/imu lpf x1 ==
  in : Inport
  "cutoff freq, Hz" : Inport  Port=2
  Filter Factor Calc : Subsystem
  Single Pole Low Pass Filter : lib_CATutils_Filters_1Pole_LowPass/Single Pole Low Pass Filter  extFactor=on  extReset=off  incIntWordSize=off  mainInternalRes=off  filtFactor=.0001
  Single Pole Low Pass Filter1 : lib_CATutils_Filters_1Pole_LowPass/Single Pole Low Pass Filter  extFactor=on  extReset=off  incIntWordSize=off  mainInternalRes=off  filtFactor=.0001
  out : Outport
  wires:
  Filter Factor Calc/1(Filter Factor) -> Single Pole Low Pass Filter/2, Single Pole Low Pass Filter1/2
  "cutoff freq, Hz"/1 -> Filter Factor Calc/1(Cutoff (Hz))
  Single Pole Low Pass Filter/1 -> Single Pole Low Pass Filter1/1
  Single Pole Low Pass Filter1/1 -> out/1
  in/1 -> Single Pole Low Pass Filter/1

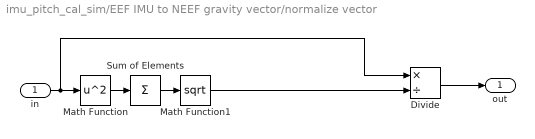
== system imu_pitch_cal_sim/EEF IMU to NEEF gravity vector/normalize vector ==
  in : Inport
  Divide : Product  Inputs=*/  OutDataTypeStr=Inherit: Same as first input
  Math Function : Math  Operator=square  SaturateOnIntegerOverflow=on
  Math Function1 : Math  Operator=sqrt  SaturateOnIntegerOverflow=on
  Sum of Elements : Sum  Inputs=+
  out : Outport
  wires:
  Sum of Elements/1 -> Math Function1/1
  Math Function/1 -> Sum of Elements/1
  Math Function1/1 -> Divide/2
  in/1 -> Divide/1, Math Function/1
  Divide/1 -> out/1

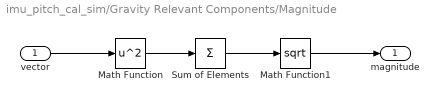
== system imu_pitch_cal_sim/Gravity Relevant Components/Magnitude ==
  vector : Inport
  Math Function : Math  Operator=square  SaturateOnIntegerOverflow=on
  Math Function1 : Math  Operator=sqrt  SaturateOnIntegerOverflow=on
  Sum of Elements : Sum  Inputs=+
  magnitude : Outport
  wires:
  Math Function1/1 -> magnitude/1
  Math Function/1 -> Sum of Elements/1
  Sum of Elements/1 -> Math Function1/1
  vector/1 -> Math Function/1

== system imu_pitch_cal_sim/Lift Cylinder Force/diameter to area ==
  diameter : Inport
  Constant2 : Constant  Value=pi/4  OutDataTypeStr=single
  Math Function : Math  Operator=square  OutputSignalType=real  SaturateOnIntegerOverflow=on
  Multiply2 : Product  SaturateOnIntegerOverflow=on  RndMeth=Zero  InputSameDT=on  OutDataTypeStr=Inherit: Same as first input
  area : Outport
  wires:
  Constant2/1 -> Multiply2/1
  Math Function/1 -> Multiply2/2
  Multiply2/1 -> area/1
  diameter/1 -> Math Function/1

== system imu_pitch_cal_sim/Lift Cylinder Force/diameter to area1 ==
  diameter : Inport
  Constant2 : Constant  Value=pi/4  OutDataTypeStr=single
  Math Function : Math  Operator=square  OutputSignalType=real  SaturateOnIntegerOverflow=on
  Multiply2 : Product  SaturateOnIntegerOverflow=on  RndMeth=Zero  InputSameDT=on  OutDataTypeStr=Inherit: Same as first input
  area : Outport
  wires:
  Constant2/1 -> Multiply2/1
  Math Function/1 -> Multiply2/2
  Multiply2/1 -> area/1
  diameter/1 -> Math Function/1

== system imu_pitch_cal_sim/Tilt Cylinder Force/diameter to area ==
  diameter : Inport
  Constant2 : Constant  Value=pi/4  OutDataTypeStr=single
  Math Function : Math  Operator=square  OutputSignalType=real  SaturateOnIntegerOverflow=on
  Multiply2 : Product  SaturateOnIntegerOverflow=on  RndMeth=Zero  InputSameDT=on  OutDataTypeStr=Inherit: Same as first input
  area : Outport
  wires:
  Constant2/1 -> Multiply2/1
  Math Function/1 -> Multiply2/2
  Multiply2/1 -> area/1
  diameter/1 -> Math Function/1

== system imu_pitch_cal_sim/Tilt Cylinder Force/diameter to area1 ==
  diameter : Inport
  Constant2 : Constant  Value=pi/4  OutDataTypeStr=single
  Math Function : Math  Operator=square  OutputSignalType=real  SaturateOnIntegerOverflow=on
  Multiply2 : Product  SaturateOnIntegerOverflow=on  RndMeth=Zero  InputSameDT=on  OutDataTypeStr=Inherit: Same as first input
  area : Outport
  wires:
  Constant2/1 -> Multiply2/1
  Math Function/1 -> Multiply2/2
  Multiply2/1 -> area/1
  diameter/1 -> Math Function/1

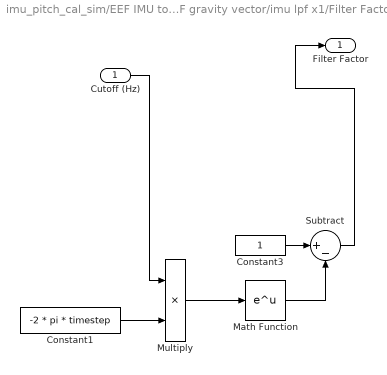
== system imu_pitch_cal_sim/EEF IMU to NEEF gravity vector/imu lpf x1/Filter Factor Calc ==
  Cutoff (Hz) : Inport
  Constant1 : Constant  Value=-2 * pi * timestep  OutDataTypeStr=single
  Constant3 : Constant  OutDataTypeStr=single
  Math Function : Math  OutputSignalType=real  SaturateOnIntegerOverflow=on
  Multiply : Product  SaturateOnIntegerOverflow=on  RndMeth=Zero  InputSameDT=on  OutDataTypeStr=Inherit: Same as first input
  Subtract : Sum  Inputs=|+-  SaturateOnIntegerOverflow=on  InputSameDT=on  OutDataTypeStr=Inherit: Same as first input
  Filter Factor : Outport
  wires:
  Constant1/1 -> Multiply/2
  Math Function/1 -> Subtract/2
  Multiply/1 -> Math Function/1
  Constant3/1 -> Subtract/1
  Subtract/1 -> Filter Factor/1
  Cutoff (Hz)/1 -> Multiply/1

== stateflow chart Chart1 ==
  state waitStart
  state raise
    en:
    calDirectionFlag = 0;
    resetRaiseFlag = 1;
    resetLowerFlag = 1;
    send(imucal)
    resetRaiseFlag = 0;
    resetLowerFlag = 0;
    du:
    send(imucal)
  state lower
    en:
    calDirectionFlag = 1;
    resetLowerFlag = 1;
    send(imucal)
    resetLowerFlag = 0;
    du:
    send(imucal)
  state endSet
    en:
    getPitchOffsetFlag = 1;
    send(imucal)
    ex:
    getPitchOffsetFlag = 0;
    calSet = 2;
  state init
    entry:
    calSet = 1
    resetRaiseFlag = 0;
    resetLowerFlag = 0;
    getPitchOffsetFlag = 0;
    calDirectionFlag = 0;
  state finalEnd
  (default) -> init
  init -> waitStart
  raise -> lower : [(calSet ==1 && time>s1c2) ||...
      | (calSet == 2 && time>s2c2)]
  waitStart -> raise : [(calSet ==1 && time>s1c1) ||...
      | (calSet == 2 && time>s2c1)]
  lower -> endSet : [(calSet ==1 && time>s1c3) ||...
      | (calSet == 2 && time>s2c3)]
  endSet -> waitStart [order 1] : [calSet == 1]
  endSet -> finalEnd [order 2] : [calSet==2]
  data: time input double; resetLowerFlag output double; resetRaiseFlag output double; calDirectionFlag output double; getPitchOffsetFlag output double; calSet local double =0; s1c1 input double; s1c2 input double; s1c3 input double; s2c1 input double; s2c2 input double; s2c3 input double
  events: imucal output FUNCTION_CALL_EVENT

== matlab function Modify IMU Pitch Orientation/Rotation Matrix About IMU neg Y axis ==
  data: angle input double; rotMatrix output double
function rotMatrix = fcn(angle)
% Calculates a rotation matrix from an angle in deg
if angle == 0
    rotMatrix = single(eye(3));
    return
end

angleRad = angle / 180.0 * pi;

% Form rotation matrix
a = cos(angleRad);
b = sin(angleRad);
rotMatrix = inv([   % Inversion to make Y rot into neg Y rot
    a, 0, b;
    0, 1, 0;
    -b, 0, a
    ]);

== matlab function EEF IMU to NEEF gravity vector/EEF vector to NEEF vector ==
  data: eefVector input double; neefVector output double; steeringAngle input double
function neefVector  = fcn(eefVector, steeringAngle)
% Transforms a vector on the EEF to a vector on the NEEF via steering angle
rotAxis = [0; 1; 0];               % Steering right is positive angle
angle = steeringAngle;

% Form rotation matrix
crossProductMatrix = [
    0,          -rotAxis(3),  rotAxis(2);
     rotAxis(3), 0,          -rotAxis(1);
    -rotAxis(2), rotAxis(1),  0
];
tensorProduct = rotAxis * transpose(rotAxis);
rotMatrix = cos(angle) * eye(3) + sin(angle) * crossProductMatrix + ...
    (1 - cos(angle)) * tensorProduct;

neefVector = rotMatrix * eefVector;

== matlab function EEF IMU to NEEF gravity vector/Rotation Matrix About Z ==
  data: angle input double; rotMatrix output double
function rotMatrix = fcn(angle)
% Calculates a rotation matrix from an angle in deg
if angle == 0
    rotMatrix = single(eye(3));
    return
end

angleRad = angle / 180.0 * pi;

% Form rotation matrix
a = cos(angleRad);
b = sin(angleRad);
rotMatrix = [
    a, -b, 0;
    b, a, 0;
    0, 0, 1
    ];

== matlab function EEF IMU to NEEF gravity vector/euler angles from rot matrix ==
  data: rotations output double; rotMatrix input double
function rotations  = decomp(rotMatrix)
%   Input:  3x3 rotation matrix
%   Output: 1x3 vector of euler angles in degrees
rotations = zeros(1,3);
rotations(1) = atan2(rotMatrix(3,2),rotMatrix(3,3));
rotations(2) = atan2(-rotMatrix(3,1), (sqrt((rotMatrix(3,2)^2)+(rotMatrix(3,3)^2))));
rotations(3) = atan2(rotMatrix(2,1),rotMatrix(1,1));
% convert back to degrees
for i=1:size(rotations,2)
    rotations(i) = 180*rotations(i)/pi;
end
end

== matlab function EEF IMU to NEEF gravity vector/rotation matrix calc from two vectors ==
  data: level_vec_meas input double; rotMatrix output double; level_vec_act input double; rotAxis output double; angle output double
function [rotMatrix, rotAxis, angle] = fcn(level_vec_meas, level_vec_act)
% Should match output of:
%     vrrotvec2mat(vrrotvec(level_vec_meas, level_vec_act))

if all(level_vec_meas == level_vec_act)
    % No transform necessary, return identity matrix
    rotAxis = single([9999; 9999; 9999]);
    angle = single(9999);
    rotMatrix = single(eye(3));
    return
end
    
a = level_vec_meas;
b = level_vec_act;

cp = cross(a, b);
cpNorm = norm(cp);

rotAxis = cp/cpNorm;
angle_rad = atan(cpNorm/dot(a, b));
angle = angle_rad * 180.0 / pi;

% Form rotation matrix
crossProductMatrix = [
    0,          -rotAxis(3),  rotAxis(2);
     rotAxis(3), 0,          -rotAxis(1);
    -rotAxis(2), rotAxis(1),  0
];
tensorProduct = rotAxis * transpose(rotAxis);
rotMatrix = cos(angle_rad) * eye(3) + sin(angle_rad) * crossProductMatrix + ...
    (1 - cos(angle_rad)) * tensorProduct;
